simulink subsystem "controladorBA"  (R2022b)
settings: Solver=VariableStepAuto  StartTime=0.0  StopTime=10.0  RelTol=1e-3
settings Model: Creator=miriamfreiriasanjuan  LastModifiedBy=miriamfreiriasanjuan

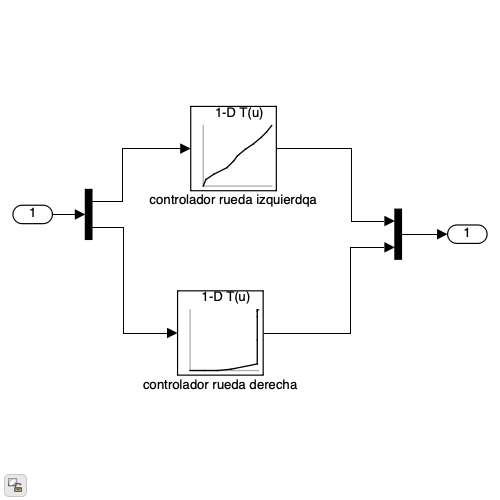
[thumbnail: Simulink's stored preview of the top-level diagram]
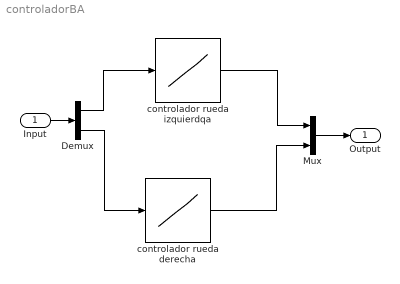
== system controladorBA ==
  Input : Inport
  Demux : Demux  Outputs=2
  Mux : Mux  Inputs=2
  controlador rueda derecha : Lookup_n-D  NumberOfTableDimensions=1  BreakpointsForDimension1=[-0.4206 -0.3418 -0.2629 -0.1709 -0.0657 0 0.1052 0.2103 0.2892 0.3681 0.4338]  Table=[-255 -200 -150 -100 -50 0 50 100 150 200 255]  InternalRulePriority=Speed  RndMeth=Simplest
  controlador rueda izquierdqa : Lookup_n-D  NumberOfTableDimensions=1  BreakpointsForDimension1=[-0.4206 -0.3812 -0.2892 -0.13 -0.0526 0 0.1052 0.1972 0.2892 0.3549 0.4206]  Table=[-255 -200 -150 -100 -50 0 50 100 150 200 255]  InternalRulePriority=Speed  RndMeth=Simplest
  Output : Outport
  wires:
  Demux/1 -> controlador rueda izquierdqa/1
  controlador rueda izquierdqa/1 -> Mux/1
  controlador rueda derecha/1 -> Mux/2
  Demux/2 -> controlador rueda derecha/1
  Input/1 -> Demux/1
  Mux/1 -> Output/1
